simulink model "simulink_motor_2025a"  (R2025a)
settings: Solver=FixedStepAuto  StartTime=0.0  StopTime=inf  RelTol=1e-3  EnableMultiTasking=on
libraries: arduinolib x3, arduinosensorlib x1
settings Model: SimulationMode=external  SILPILModeSetting=veronly  ExtModeTrigDuration=2  Creator=Kleiton  LastModifiedBy=Kleiton
settings SolverCC: AutoInsertRateTranBlk=on
settings OptimizationCC: EnhancedBackFolding=on  PassReuseOutputArgsAs=Individual arguments  ZeroExternalMemoryAtStartup=off  ZeroInternalMemoryAtStartup=off  MaxStackSize=64  OptimizeBlockOrder=speed  DifferentSizesBufferReuse=on  OptimizationCustomize=off  EfficientTunableParamExpr=on
settings DebuggingCC: ParameterTunabilityLossMsg=error
settings HardwareCC: ProdBitPerInt=16.0  ProdBitPerPointer=16.0  ProdBitPerSizeT=16.0  ProdBitPerPtrDiffT=16.0  ProdLargestAtomicFloat=None  ProdWordSize=8.0  ProdHWDeviceType=Atmel->AVR
settings SFSimCC: MATLABDynamicMemAlloc=off
settings RTWCC: SystemTargetFile=ert.tlc  HardwareBoard=Arduino Uno  TemplateMakefile=ert_default_tmf  Toolchain=Arduino AVR  BuildConfiguration=Faster Runs  Description=Embedded Coder
settings CodeAppCC: ForceParamTrailComments=on  IgnoreCustomStorageClasses=off  OperatorAnnotations=on  SimulinkDataObjDesc=on  SFDataObjDesc=on  InsertBlockDesc=on
settings ERTTargetCC: ExtModeTransport=3.0  ExtModeAutomaticAllocSize=off  ExtModeStaticAllocSize=250.0  InlinedParameterPlacement=Hierarchical  SupportContinuousTime=on  SupportVariableSizeSignals=on

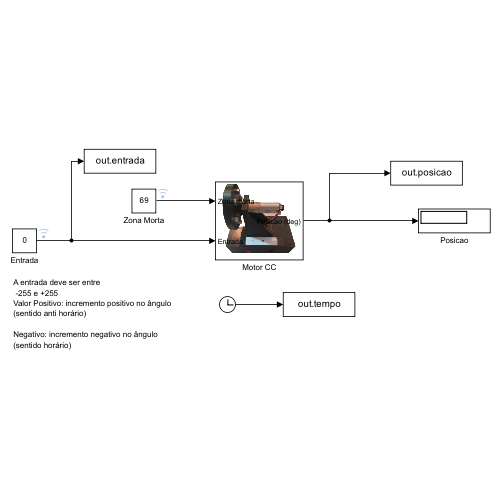
[thumbnail: Simulink's stored preview of the top-level diagram]
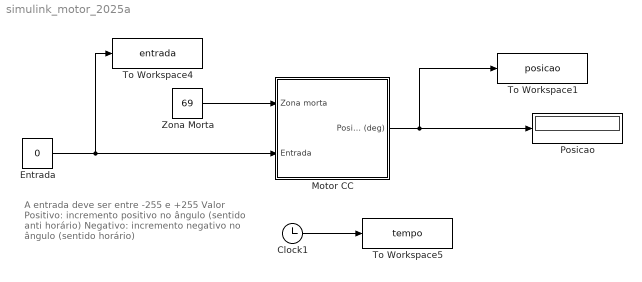
== system simulink_motor_2025a ==
  note: A entrada deve ser entre
      |  -255 e +255
      | Valor Positivo: incremento positivo no ângulo
      | (sentido anti horário)
      |
      | Negativo: incremento negativo no ângulo
      | (sentido horário)
  Clock1 : Clock
  Entrada : Constant  Value=0
  Motor CC : Subsystem
      mask Display: image('motor_cc.png');
  Posicao : Display
  To Workspace1 : ToWorkspace  VariableName=posicao  SampleTime=-1
      settings: Save2DSignal=2-D array (concatenate along first dimension)
  To Workspace4 : ToWorkspace  VariableName=entrada  SampleTime=-1
      settings: Save2DSignal=2-D array (concatenate along first dimension)
  To Workspace5 : ToWorkspace  VariableName=tempo  SampleTime=-1
      settings: Save2DSignal=2-D array (concatenate along first dimension)
  Zona Morta : Constant  Value=69
  wires:
  Entrada/1 -> Motor CC/2(Entrada), To Workspace4/1
  Motor CC/1(Posicao (deg)) -> Posicao/1, To Workspace1/1
  Clock1/1 -> To Workspace5/1
  Zona Morta/1 -> Motor CC/1(Zona morta)

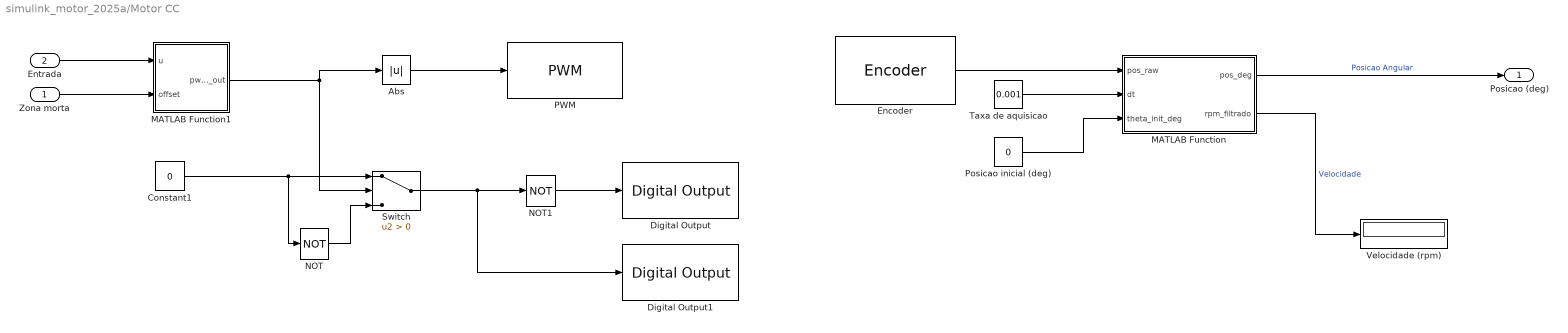
== system simulink_motor_2025a/Motor CC ==
  Zona morta : Inport
  Entrada : Inport  Port=2
  Abs : Abs  SaturateOnIntegerOverflow=off
  Constant1 : Constant  Value=0
  Digital Output : arduinolib/Digital Output  pinNumber=8  Direction=output  blockPlatform=arduino
  Digital Output1 : arduinolib/Digital Output  pinNumber=7  Direction=output  blockPlatform=arduino
  Encoder : arduinosensorlib/Encoder  InputA=2  InputB=3  Mode=No reset  SampleTime=0.001
  MATLAB Function : MATLAB Function  TreatAsAtomicUnit=on
  MATLAB Function1 : MATLAB Function  TreatAsAtomicUnit=on
  NOT : Logic  Operator=NOT  IconShape=distinctive  AllPortsSameDT=off  OutDataTypeStr=boolean
  NOT1 : Logic  Operator=NOT  IconShape=distinctive  AllPortsSameDT=off  OutDataTypeStr=boolean
  PWM : arduinolib/PWM  pinNumber=11  frequencyType=Specify  desiredFrequency=3921.16  achievableFrequency=3921.16
  Posicao inicial (deg) : Constant  Value=0
  Switch : Switch  Criteria=u2 > Threshold  SaturateOnIntegerOverflow=off  InputSameDT=off
  Taxa de aquisicao : Constant  Value=0.001
  Velocidade (rpm) : Display
  Posicao (deg) : Outport
  wires:
  Zona morta/1 -> MATLAB Function1/2(offset)
  Switch/1 -> Digital Output1/1, NOT1/1
  MATLAB Function/1(pos_deg) -> Posicao (deg)/1  "Posicao Angular"
  MATLAB Function1/1(pwm_out) -> Abs/1, Switch/2
  Taxa de aquisicao/1 -> MATLAB Function/2(dt)
  Entrada/1 -> MATLAB Function1/1(u)
  Posicao inicial (deg)/1 -> MATLAB Function/3(theta_init_deg)
  NOT1/1 -> Digital Output/1
  Abs/1 -> PWM/1
  Encoder/1 -> MATLAB Function/1(pos_raw)
  MATLAB Function/2(rpm_filtrado) -> Velocidade (rpm)/1  "Velocidade"
  Constant1/1 -> NOT/1, Switch/1
  NOT/1 -> Switch/3

== matlab function simulink_motor_2025a/Motor CC/MATLAB Function ==
  data: pos_raw input; pos_deg output; dt input; rpm_filtrado output; theta_init_deg input
function [pos_deg, rpm_filtrado] = fcn(pos_raw, dt, theta_init_deg)
    % Converte entradas para double para evitar estouro/incompatibilidade de tipos
    pos = double(pos_raw);
    theta_init = double(theta_init_deg); % Ângulo inicial em graus
    
    % Variáveis persistentes para histórico entre amostras
    persistent offset pos_anterior rpm_anterior is_initialized;
    
    % 1. Parâmetros do Motor GA25-370 (Redução 1:46.85)
    ppr_motor = 11;                          % Pulsos nativos do disco magnético
    cpr_simulink = ppr_motor * 4;            % Quadratura 4x do Simulink (44 contagens/volta)
    reducao_caixa = 46.85;                   % Redução mecânica interna da caixa
    
    cpr_saida = cpr_simulink * reducao_caixa; % 2061.4 contagens por volta completa na saída
    
    % 2. Inicialização na primeira execução (t = 0)
    if isempty(is_initialized)
        offset = pos;
        pos_anterior = theta_init; % Posição inicial do histórico em graus
        rpm_anterior = 0;          % RPM filtrado do ciclo anterior
        is_initialized = true;
    end
    
    % 3. Posição Angular em Graus (Saída do Motor + Offset Inicial)
    pulsos_relativos = pos - offset;
    pos_deg = (pulsos_relativos * (360 / cpr_saida)) + theta_init;
    
    % 4. Velocidade Instantânea em RPM (Derivada Discreta baseada em Graus)
    if dt > 0
        d_deg = pos_deg - pos_anterior;
        % Conversão: (deg / dt) * (1 volta / 360 deg) * (60 s / 1 min) = RPM
        rpm_raw = (d_deg / dt) * (60 / 360);
    else
        rpm_raw = 0;
    end
    
    % 5. Filtro Passa-Baixas Exponencial (IIR de 1ª Ordem)
    fc = 5.0; % Frequência de corte em Hz
    tau = 1 / (2 * pi * fc);
    alpha = dt / (tau + dt); % Fator de suavização proporcional a dt
    
    rpm_filtrado = alpha * rpm_raw + (1 - alpha) * rpm_anterior;
    
    % 6. Atualiza as variáveis para a próxima amostragem
    pos_anterior = pos_deg;
    rpm_anterior = rpm_filtrado;
end

== matlab function simulink_motor_2025a/Motor CC/MATLAB Function1 ==
  data: u input; pwm_out output; offset input
function pwm_out = compensador_avancado(u, offset)
    limiar = 0; % Margem para ignorar ruído em torno de zero

    if u > limiar
        pwm_out = u + offset;
    elseif u < -limiar
        pwm_out = u - offset;
    else
        pwm_out = 0; % Não ativa o motor para ruídos residuais
    end

    % Saturação do sinal de saída para o limite do PWM (-255 a 255)
    pwm_out = min(max(pwm_out, -255), 255);
end
